simulink model "pmsm_with_fuel_cell"  (R2024b)
settings: Solver=ode14x  StartTime=0.0  StopTime=1  MaxStep=2e-6  RelTol=1e-3
InitFcn:
  | % Control parameters
  | Ts = 2e-6;   % Fundamental sample time
  | fsw = 2e3;   % Switching frequency (Hz)
  | fc = fsw*10; % Control loop frequency (Hz)
  | Tsc = 1/fc;  % Control loop sample time
  | 
  | % PMSM parameters
  | PM = 0.03; % Permanent magnet flux linkage
  | Ld = 2e-4;  % d-axis inductance
  | Lq = 2e-4;  % q-axis inductance
  | L0 = 2e-4;  % 0-axis inductance
  | Rs = 0.013; % Stator resistance
  | N = 6; % Number of pole pairs
  | J = 0.2; % Moment of inertia
  | 
  | % Operating and derived limits
  | Imax = 100;  % Max stator current (peak value)
  | Tmax = 1.5*N*PM*Imax; % Max lectromagnetic torque
  | fnom = 100;  % Nominal frequency (Hz)
  | rpm_nom = 60*fnom/N;      % Nominal rotor speed (rpm)
  | omegam_nom = 2*pi*fnom/N; % Nominal mechanical rotor speed
  | Pmax = omegam_nom*Tmax;     % Maximum power
libraries: fl_lib x27, nesl_utility x24, ee_lib x18, batteryecm_lib x1, eePmsmFieldOrientedControl x1, rllib x1
(part 1 of 2)
settings Model: SimulationMode=accelerator  Creator=pruth  LastModifiedBy=pruth
settings SolverCC: ExtrapolationOrder=2
settings DebuggingCC: SignalInfNanChecking=error
settings SimscapeCC: SimscapeLogType=all

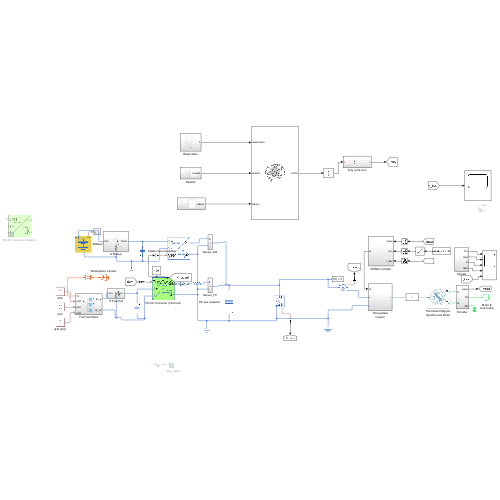
[thumbnail: Simulink's stored preview of the top-level diagram]
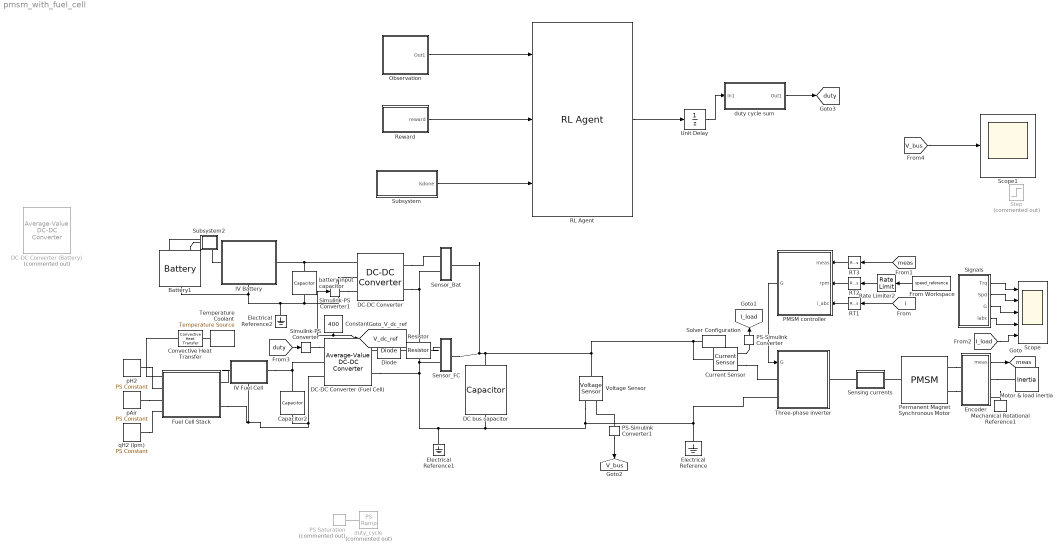
== system pmsm_with_fuel_cell ==
  Battery1 : batteryecm_lib/Battery  Vnom=400 V  prm_dir=1  R1_dis=2 Ohm  R1_ch=2 Ohm  R1=0.05 Ohm  prm_AH=2  AH=30 hr*A  V1=330 V  AH1=15 hr*A  prm_R2=1  R2=2000 Ohm  Tmeas=298.15 K  charge_measurement_port=simscape.enum.battery.enable.yes  prm_dyn=1  Rp1=0.005 Ohm  tau1=30 s  Rp2=0.005 Ohm  tau2=30 s  Rp3=0.005 Ohm  tau3=30 s  Rp4=0.005 Ohm  tau4=30 s  Rp5=0.005 Ohm  tau5=30 s  prm_fade=simscape.enum.battery.prm_fade.enabled  N_fade=10000  AH_fade=29.7 hr*A  R1_fade=0.0505 Ohm  R1_ch_fade=2.02 Ohm  V1_fade=329 V  prm_age=1  prm_age_OCV=1  OCV_age=0.9  SOC_age=60  Tmeas_age=298.15 K  delta_time_age_vec=[0] d  temperature_age_vec=[273] K  OCV_scaling_age=2.2134e6  OCV_offset_age=1.632e6  temp_exp_age=0.515833569 V  t_exp_age=0.75  Vnom_T2=12 V  R1_T2=2.2 Ohm  R1_T2_dis=2.2 Ohm  R1_T2_ch=2.2 Ohm  V1_T2=11.4 V  R2_T2=2200 Ohm  Rp1_T2=0.005 Ohm  tau1_T2=30 s  Rp2_T2=0.005 Ohm  tau2_T2=30 s  Rp3_T2=0.005 Ohm  tau3_T2=30 s  Rp4_T2=0.005 Ohm  tau4_T2=30 s  Rp5_T2=0.005 Ohm  tau5_T2=30 s  Tmeas2=273.15 K  thermal_port=simscape.enum.thermaleffects.omit  thermal_mass=30000 J/K  i_specify=off  i_priority=None  i=0 A  i_nominal_specify=off  i_nominal_value=1  i_nominal_unit=A  v_specify=on  v_priority=Low  v=330 V  v_nominal_specify=off  v_nominal_value=1  v_nominal_unit=V  charge_specify=on  charge_priority=High  charge=15 hr*A  charge_nominal_specify=off  charge_nominal_value=1  charge_nominal_unit=hr*A  num_cycles_specify=on  num_cycles_priority=High  num_cycles=10  num_cycles_nominal_specify=off  num_cycles_nominal_value=1  num_cycles_nominal_unit=1  temperature_specify=off  temperature_priority=High  temperature=298.15 K  temperature_nominal_specify=off  temperature_nominal_value=1  temperature_nominal_unit=K
      settings: LogSimulationData=on  InternalSimscapePortConfiguration="{\"Bottom\":[],\"Left\":[{\"id\":\"p\",\"label\":\"+\",\"type\":\"foundation.electrical.electrical\"},{\"id\":\"q\",\"label\":\"q\",\"type\":\"output\"}],\"Right\":[{\"id\":\"n\",\"label\":\"-\",\"type\":\"foundation.electrical.electrical\"}],\"Top\":[]}"
  Capacitor2 : fl_lib/Electrical/Electrical Elements/Capacitor  c=1e-3 F  r=1e-3 Ohm  g=0 1/Ohm  i_specify=off  i_priority=None  i=0 A  i_nominal_specify=off  i_nominal_value=1  i_nominal_unit=A  v_specify=off  v_priority=None  v=0 V  v_nominal_specify=off  v_nominal_value=1  v_nominal_unit=V  vc_specify=on  vc_priority=Low  vc=650 V  vc_nominal_specify=off  vc_nominal_value=1  vc_nominal_unit=V
  Constant : Constant  Value=400
  Convective Heat Transfer : fl_lib/Thermal/Thermal Elements/Convective Heat Transfer  thermal_type=foundation.enum.constant_variable.constant  area=300 cm^2  heat_tr_coeff=75 W/(m^2 * K)  min_heat_tr_coeff=1e-3 W/(K*m^2)  T_specify=off  T_priority=None  T=0 K  T_nominal_specify=off  T_nominal_value=1  T_nominal_unit=K  Q_specify=off  Q_priority=None  Q=0 W  Q_nominal_specify=off  Q_nominal_value=1  Q_nominal_unit=W
  Current Sensor : fl_lib/Electrical/Electrical Sensors/Current Sensor
  DC bus capacitor : fl_lib/Electrical/Electrical Elements/Capacitor  c=5 mF  r=1e-3 Ohm  g=0 1/Ohm  i_specify=off  i_priority=None  i=0 A  i_nominal_specify=off  i_nominal_value=1  i_nominal_unit=A  v_specify=off  v_priority=Low  v=400 V  v_nominal_specify=off  v_nominal_value=1  v_nominal_unit=V  vc_specify=on  vc_priority=High  vc=400 V  vc_nominal_specify=off  vc_nominal_value=1  vc_nominal_unit=V
  DC-DC Converter : ee_lib/Semiconductors & Converters/Converters/DC-DC Converter  Vref_option=ee.enum.converters.voltageref.external  v_ref=10 V  P_rated=10000 W  droop_enabled=true  droop_param=ee.enum.converters.droop.value  droop=0.15 V/A  droop_percent=2  Vref_droop=400 V  reversible=ee.enum.converters.directionality.bidirectional  G_diode=1e-8 1/Ohm  P_fixed=0.5 W  losses_option=ee.enum.converters.lossesOption.proportionalToSquaredCurrent  eff_rated=98  tableOption=ee.enum.converters.lossTableOptionThermal.currentTemp  i_eff_vec=[-2, -1, 1, 2] A  v_eff_vec=[15, 30, 45] V  eff_vec=[66, 76, 80, 74]  eff_2D_table=[66, 66, 66; 76, 76, 76; 80, 80, 80; 74, 74, 74]  model_dynamics=ee.enum.converters.dynamics.no  tau=0.005 s  v_ini=400 V  v1_min=1 V  R1=1000 Ohm  R2=1000 Ohm  fault_condition=ee.enum.faults.faultInputCondition.greaterThan  fault_threshold=0.5  T_eff_vec=[280, 300, 320] K  eff_3D_table=repmat([66; 76; 80; 74], 1, 3, 3)  thermal_mass=100 J/K  initial_temperature=298.15 K
      settings: InternalSimscapePortConfiguration="{\"Bottom\":[],\"Left\":[{\"id\":\"p1\",\"label\":\"1+\",\"type\":\"foundation.electrical.electrical\"},{\"id\":\"n1\",\"label\":\"1-\",\"type\":\"foundation.electrical.electrical\"},{\"id\":\"Vref\",\"label\":\"Vref\",\"type\":\"input\"}],\"Right\":[{\"id\":\"p2\",\"label\":\"2+\",\"type\":\"foundation.electrical.electrical\"},{\"id\":\"n2\",\"label\":\"2-\",\"type\":\"foundation.electrical.electrical\"}],\"Top\":[]}"
  DC-DC Converter (Battery) : ee_lib/Semiconductors & Converters/Converters/Average-Value DC-DC Converter  Commented=on  control_option=ee.enum.converters.controlinput.voltage  converter_type=ee.enum.converters.dcdctype.boost  efficiency_option=ee.enum.converters.efficiency.constant  efficiency_fixed=100  i_vec=[0, 2, 5] A  efficiency_vec=[90, 95, 98]
      settings: LogSimulationData=on  InternalSimscapePortConfiguration="{\"Bottom\":[],\"Left\":[{\"id\":\"Vref\",\"label\":\"Vref\",\"type\":\"input\"},{\"id\":\"p1\",\"label\":\"1+\",\"type\":\"foundation.electrical.electrical\"},{\"id\":\"n1\",\"label\":\"1-\",\"type\":\"foundation.electrical.electrical\"}],\"Right\":[{\"id\":\"p2\",\"label\":\"2+\",\"type\":\"foundation.electrical.electrical\"},{\"id\":\"n2\",\"label\":\"2-\",\"type\":\"foundation.electrical.electrical\"}],\"Top\":[]}"
  DC-DC Converter (Fuel Cell) : ee_lib/Semiconductors & Converters/Converters/Average-Value DC-DC Converter  control_option=ee.enum.converters.controlinput.dutycycle  converter_type=ee.enum.converters.dcdctype.buck  efficiency_option=ee.enum.converters.efficiency.constant  efficiency_fixed=100  i_vec=[0, 2, 5] A  efficiency_vec=[90, 95, 98]
      settings: LogSimulationData=on  InternalSimscapePortConfiguration="{\"Bottom\":[],\"Left\":[{\"id\":\"DutyCycle\",\"label\":\"DutyCycle\",\"type\":\"input\"},{\"id\":\"p1\",\"label\":\"1+\",\"type\":\"foundation.electrical.electrical\"},{\"id\":\"n1\",\"label\":\"1-\",\"type\":\"foundation.electrical.electrical\"}],\"Right\":[{\"id\":\"p2\",\"label\":\"2+\",\"type\":\"foundation.electrical.electrical\"},{\"id\":\"n2\",\"label\":\"2-\",\"type\":\"foundation.electrical.electrical\"}],\"Top\":[]}"
  Diode : ee_lib/Semiconductors & Converters/Diode  ModelType=ee.enum.diode.modelType.pwl  TableType=ee.enum.diode.tableType.IfMat  IfMat=[.07, .12, .19, 1.75, 4.24, 7.32, 11.2; .16, .3, .72, 2.14, 5.02, 8.35, 13.12] A  VfMat=[.9, 1.15, 1.25, 1.5, 1.75, 2.17, 2.6, 2.85; .58, .68, .75, 1.1, 1.38, 1.77, 2.27, 2.7] V  TjVec=[25, 125] degC  VfVec=[.5, .7, .9, 1.3, 1.7, 2.1, 2.5] V  IfVec=[.1, .2, .5, 1, 2, 4, 7, 10] A  IrMat=[1e-06, 2e-06, 5e-06, 1e-05, 2.5e-05, 5e-05, .0001; 2e-06, 5e-06, 1e-05, 4e-05, 8e-05, .0002, .0005] A  VrMat=[10, 100, 200, 250, 300, 325, 350; 10, 70, 160, 220, 270, 300, 320] V  VrVec=[10, 20, 40, 50, 70, 80, 100] V  IrVec=[1e-06, 2e-06, 5e-06, 1e-05, 2e-05, 5e-05, .0001] A  Vf=0.8 V  Ron=0.001 Ohm  Goff=1e-8 S  prmExp=ee.enum.diode.expParam.useTwo  I12=[.0137, .545] A  V12=[.6, .7] V  RS=0 Ohm  Tmeas=298.15 K  IS=1e-12 A  ec=1  I1=0.0137 A  V1=0.6 V  N_series=1  N_parallel=1  ZenerEnable=false  Rz=0.3 Ohm  BV=inf V  C_param=ee.enum.diode.capParam.fixed  CJ=0 pF  CJ0=5 pF  Vvec=[.1, 10, 100] V  Cvec=[3.5, 1, .4] pF  VJ=1 V  Mgrad=0.5  FC=0.5  Q_param=ee.enum.diode.recoveryParam.off  iRM=-7.15 A  iF=4 A  didt=-750 A/us  trr_factor=3  trr=115 ns  Qrr=150 nA*s  Vr=-600 V  Ls=150 nH  Erec=0.03 J  TT=50 ns  tau=100 ns  T_param=ee.enum.diode.temperatureParam.off  Tdevice=298.15 K  I1_T2=0.245 A  V1_T2=0.5 V  IS_T2=1.25e-7 A  Tmeas2=125 degC  XTI_param=ee.enum.diode.xtiParam.pn  XTI=3  EG_param=ee.enum.diode.egapParam.material_si  EG=1.11 eV  dBVdT=0 V/K  fault_action=simscape.enum.assert.action.none  t_fault=inf s  enable_fault_input=simscape.enum.onoff.off  i_specify=off  i_priority=None  i=0 A  i_nominal_specify=off  i_nominal_value=1  i_nominal_unit=A  v_specify=off  v_priority=None  v=0 V  v_nominal_specify=off  v_nominal_value=1  v_nominal_unit=V  v_capacitor_specify=off  v_capacitor_priority=None  v_capacitor=0 V  v_capacitor_nominal_specify=off  v_capacitor_nominal_value=1  v_capacitor_nominal_unit=V  Qj_specify=off  Qj_priority=High  Qj=0 C  Qj_nominal_specify=off  Qj_nominal_value=1  Qj_nominal_unit=C  i_diode_specify=off  i_diode_priority=None  i_diode=0 A  i_diode_nominal_specify=off  i_diode_nominal_value=1  i_diode_nominal_unit=A  v_diode_specify=off  v_diode_priority=None  v_diode=0 V  v_diode_nominal_specify=off  v_diode_nominal_value=1  v_diode_nominal_unit=V  i_capacitor_specify=off  i_capacitor_priority=None  i_capacitor=0 A  i_capacitor_nominal_specify=off  i_capacitor_nominal_value=1  i_capacitor_nominal_unit=A  power_dissipated_specify=off  power_dissipated_priority=None  power_dissipated=0 W  power_dissipated_nominal_specify=off  power_dissipated_nominal_value=1  power_dissipated_nominal_unit=W  fidelity_level=ee.enum.diode.fidelity.idealSwitch  rec_loss_model=ee.enum.diode.reverseRecoveryModel.fixed  ErecVal=0 J  scaleWithIandV=true  ErecMat=zeros(2, 3) J  TjrecVec=[298.15, 398.15] K  IfrecVec=[.1, 1, 10] A  IrecVal=10 A  VrecVal=10 V  tFilter=1 / 1000 / 100 s  thermal_network_parameterization=ee.enum.thermalNetworkTopology.junctionCase  Rth=[0, 10] K/W  Rth_Cauer=[1, 3, 10] K/W  Rth_Foster=[.08, .14, .22, .16] K/W  thermal_mass_parameterization=ee.enum.thermalNetwork.timeconstant  thermal_mass=[0, 1] J/K  thermal_mass_Cauer=[.1, .3, 1] J/K  thermal_mass_Foster=[.001, .005, .05, .5] J/K  thermal_time_constant=[0, 10] s  thermal_time_constant_Cauer=[1, 3, 10] s  thermal_time_constant_Foster=[7e-05, .0007, .01, .08] s  thermal_mass_initial_temperatures=[25, 25] degC  thermal_mass_initial_temperatures_Cauer=[25, 25, 25] degC  junction_thermal_mass=0.01 J/K  Tvec_initial_Foster=[25, 25, 25, 25] degC  no_thermal_network=1  junction_temperature_specify=off  junction_temperature_priority=None  junction_temperature=25 degC  junction_temperature_nominal_specify=off  junction_temperature_nominal_value=1  junction_temperature_nominal_unit=degC
  Electrical Reference : fl_lib/Electrical/Electrical Elements/Electrical Reference
  Electrical Reference1 : fl_lib/Electrical/Electrical Elements/Electrical Reference
  Electrical Reference2 : fl_lib/Electrical/Electrical Elements/Electrical Reference
  Encoder : Subsystem
  From Workspace : FromWorkspace  VariableName=speed_reference
  Fuel Cell Stack : Subsystem
  IV Battery : Subsystem
      settings: PortSchema="{\"entries\":[{\"content\":{\"sides\":[{\"content\":{\"connectorIds\":[\"LConn1\"]},\"type\":\"ConnectorPlacement.EquallySpacedRectSide\",\"uuid\":\"c74c3ffe-4181-439f-8f63-47f39e558e2a\"},{\"content\":{\"connectorIds\":[\"RConn1\"],\"side\":\"RIGHT\"},\"type\":\"ConnectorPlacement.EquallySpacedRectSide\",\"uuid\":\"9438a85a-aa2d-46a8-960b-411a29715dec\"},{\"content\":{\"side\":\"TOP\"},\"type\":\"ConnectorPlacement.EquallySpacedRectSide\",\"uuid\":\"d1231007-950c-459e-80d3-fa3ee648e50c\"},{\"content\":{\"connectorIds\":[\"RConn2\"],\"side\":\"BOTTOM\"},\"type\":\"ConnectorPlacement.EquallySpacedRectSide\",\"uuid\":\"ff976e01-1be4-46b4-8cbd-cb7b347558a5\"}]},\"type\":\"ConnectorPlacement.EquallySpacedConnector\",\"uuid\":\"65ee485a-61b0-4423-8d03-0ee370ce5677\"}],\"packageUris\":[\"http://schema.mathworks.com/mf0/Connector/R2020b\"],\"version\":\"1.0\"}"
  IV Fuel Cell : Subsystem
      settings: PortSchema="{\"entries\":[{\"content\":{\"sides\":[{\"content\":{\"connectorIds\":[\"LConn1\"]},\"type\":\"ConnectorPlacement.EquallySpacedRectSide\",\"uuid\":\"c74c3ffe-4181-439f-8f63-47f39e558e2a\"},{\"content\":{\"connectorIds\":[\"RConn1\"],\"side\":\"RIGHT\"},\"type\":\"ConnectorPlacement.EquallySpacedRectSide\",\"uuid\":\"9438a85a-aa2d-46a8-960b-411a29715dec\"},{\"content\":{\"side\":\"TOP\"},\"type\":\"ConnectorPlacement.EquallySpacedRectSide\",\"uuid\":\"d1231007-950c-459e-80d3-fa3ee648e50c\"},{\"content\":{\"connectorIds\":[\"RConn2\"],\"side\":\"BOTTOM\"},\"type\":\"ConnectorPlacement.EquallySpacedRectSide\",\"uuid\":\"02f3766e-517b-4ca7-9ef5-b22112c4fb5b\"}]},\"type\":\"ConnectorPlacement.EquallySpacedConnector\",\"uuid\":\"65ee485a-61b0-4423-8d03-0ee370ce5677\"}],\"packageUris\":[\"http://schema.mathworks.com/mf0/Connector/R2020b\"],\"version\":\"1.0\"}"
  Mechanical Rotational Reference1 : fl_lib/Mechanical/Rotational Elements/Mechanical Rotational Reference
  Motor & load inertia : fl_lib/Mechanical/Rotational Elements/Inertia  inertia=J kg*m^2  num_ports=foundation.enum.numPorts2.one  w_specify=on  w_priority=High  w=0 rpm  w_nominal_specify=off  w_nominal_value=1  w_nominal_unit=rad/s  t_specify=off  t_priority=High  t=0 N*m  t_nominal_specify=off  t_nominal_value=1  t_nominal_unit=N*m
  Observation : Subsystem
  PMSM controller : Subsystem
  PS Saturation : fl_lib/Physical Signals/Nonlinear Operators/PS Saturation  Commented=on  upper_limit=0.95  lower_limit=0.15
  PS-Simulink Converter : nesl_utility/PS-Simulink Converter  PhysicalDomain=network_engine_domain  SubClassName=ps_output  LeftPortType=input  RightPortType=output  PseudoPeriodic=off  Frequencies=[]  VectorFormat=inherit  Unit=inherit  AffineConversion=off
  PS-Simulink Converter1 : nesl_utility/PS-Simulink Converter  PhysicalDomain=network_engine_domain  SubClassName=ps_output  LeftPortType=input  RightPortType=output  PseudoPeriodic=off  Frequencies=[]  VectorFormat=inherit  Unit=inherit  AffineConversion=off
  Permanent Magnet Synchronous Motor : ee_lib/Electromechanical/Permanent Magnet/PMSM  port_option=ee.enum.threePhasePort.composite  winding_type=ee.enum.statorconnection.wye  machine_param=ee.enum.pmsm.parameterization.constant  nPolePairs=N  pmflux_param=ee.enum.pmflux.fluxlinkage  pm_flux_linkage=PM Wb  torque_constant=0.18 N*m/A  back_emf_constant=0.18 V/(rad/s)  stator_param=ee.enum.statorparam.LdLqL0  Ld=Ld H  Lq=Lq H  idVec=[-200, 0, 200] A  iqVec=[-200, 0, 200] A  LdMatrix=0.0002 * ones(3, 3) H  LqMatrix=0.0002 * ones(3, 3) H  PmMatrix=0.1 * ones(3, 3) Wb  ktMatrix=0.18 * ones(3, 3) N*m/A  keMatrix=0.18 * ones(3, 3) V/(rad/s)  L0=L0 H  Ls=0.0002 H  Lm=0.00002 H  Ms=0.00002 H  Rs=Rs Ohm  zero_sequence=ee.enum.park.zerosequence.exclude  axes_param=ee.enum.rotorangle.qaxis  loss_param=ee.enum.ironloss.none  losses_oc=[0, 0, 0] W  losses_sc=[0, 0, 0] W  f_losses=60 Hz  Isc_losses=95 A  J=0 kg*m^2  lam=1e-3 N*m/(rad/s)  i_d_specify=off  i_d_priority=None  i_d=0 A  i_d_nominal_specify=off  i_d_nominal_value=1  i_d_nominal_unit=A  i_q_specify=off  i_q_priority=None  i_q=0 A  i_q_nominal_specify=off  i_q_nominal_value=1  i_q_nominal_unit=A  torque_specify=off  torque_priority=None  torque=0 N*m  torque_nominal_specify=off  torque_nominal_value=1  torque_nominal_unit=N*m  angular_velocity_specify=on  angular_velocity_priority=None  angular_velocity=0 rpm  angular_velocity_nominal_specify=off  angular_velocity_nominal_value=1  angular_velocity_nominal_unit=rpm  angular_position_specify=on  angular_position_priority=High  angular_position=0 rad  angular_position_nominal_specify=off  angular_position_nominal_value=1  angular_position_nominal_unit=deg  alpha=3.93e-3 1/K  alpha_flux=-0.001 1/K  Tmeas=298.15 K  stator_thermal_mass=100 J/K  rotor_thermal_mass=200 J/K  Rm_percent_rotor=90  Rd_percent_rotor=30  temperatureA_specify=off  temperatureA_priority=High  temperatureA=25 degC  temperatureA_nominal_specify=off  temperatureA_nominal_value=1  temperatureA_nominal_unit=degC  temperatureB_specify=off  temperatureB_priority=High  temperatureB=25 degC  temperatureB_nominal_specify=off  temperatureB_nominal_value=1  temperatureB_nominal_unit=degC  temperatureC_specify=off  temperatureC_priority=High  temperatureC=25 degC  temperatureC_nominal_specify=off  temperatureC_nominal_value=1  temperatureC_nominal_unit=degC  temperatureR_specify=off  temperatureR_priority=High  temperatureR=25 degC  temperatureR_nominal_specify=off  temperatureR_nominal_value=1  temperatureR_nominal_unit=degC
      settings: InternalSimscapePortConfiguration="{\"Bottom\":[],\"Left\":[{\"id\":\"N\",\"label\":\"~\",\"type\":\"foundation.electrical.three_phase\"}],\"Right\":[{\"id\":\"R\",\"label\":\"R\",\"type\":\"foundation.mechanical.rotational.rotational\"},{\"id\":\"C\",\"label\":\"C\",\"type\":\"foundation.mechanical.rotational.rotational\"}],\"Top\":[]}"
  RL Agent : rllib/RL Agent  Agent=agent  ExternalActionAsInput=off  ProvideLastAction=off  ProvideCumRwd=off  TreatAsDirectFeedthrough=on  UseStrictObservationDataTypes=off
  RT1 : RateTransition  OutPortSampleTime=Tsc
  RT2 : RateTransition  OutPortSampleTime=Tsc
  RT3 : RateTransition  OutPortSampleTime=Tsc
  Rate Limiter2 : RateLimiter  RisingSlewLimit=8000  FallingSlewLimit=-8000  SampleTimeMode=inherited
  Resistor : fl_lib/Electrical/Electrical Elements/Resistor  R=0.1 Ohm  i_specify=off  i_priority=None  i=0 A  i_nominal_specify=off  i_nominal_value=1  i_nominal_unit=A  v_specify=off  v_priority=None  v=0 V  v_nominal_specify=off  v_nominal_value=1  v_nominal_unit=V
  Reward : Subsystem
  Scope : Scope  NumInputPorts=5
  Scope1 : Scope
  Sensing currents : Subsystem
      mask Display: disp('i')
  Sensor_Bat : Subsystem
  Sensor_FC : Subsystem
  "Signals " : Subsystem
  Simulink-PS Converter : nesl_utility/Simulink-PS Converter  PhysicalDomain=network_engine_domain  SubClassName=ps_input  LeftPortType=input  RightPortType=output  PseudoPeriodic=off  Frequencies=[]  NoiseDistribution=none  NoiseParameters=[]  Unit=1  AffineConversion=off  FilteringAndDerivatives=filter  SimscapeFilterOrder=2  InputFilterTimeConstant=1e-5  UdotUserProvided=0
  Simulink-PS Converter1 : nesl_utility/Simulink-PS Converter  PhysicalDomain=network_engine_domain  SubClassName=ps_input  LeftPortType=input  RightPortType=output  PseudoPeriodic=off  Frequencies=[]  NoiseDistribution=none  NoiseParameters=[]  Unit=1  AffineConversion=off  FilteringAndDerivatives=provide  SimscapeFilterOrder=1  InputFilterTimeConstant=0.001  UdotUserProvided=0
  Solver Configuration : nesl_utility/Solver Configuration  PhysicalDomain=network_engine_domain  SubClassName=solver  LeftPortType=input  RightPortType=generic  Tones=[]  Harmonics=[]  SimulateNoise=off  Profile=off  UseLocalSampling=off  EnableSwitchedLinearOptims=on  FrequencyDomain=off  UseCCode=off  RelTol=0.001  AbsTol=1e-06  MinStep=1e-09  ToWorkspace=off  RevertToSquareIcSolve=off  NumHomotopyIterations=100  PhasorMode=off  PhasorModeNumHarmonics=1  ConsistencySolver=NEWTON_FTOL  IndexReductionMethod=DerivativeReplacement  DoDC=off  ResidualTolerance=1e-3  ConsistencyTolSource=GLOBAL  ConsistencyAbsTol=0.001  ConsistencyRelTol=0.001  ConsistencyTolFactor=0.001  UseLocalSolver=on  LocalSolverChoice=NE_BACKWARD_EULER_ADVANCER  ResolveIndetEquations=on  FunctionEvalNumThread=1  LocalSolverSampleTime=Ts  DoFixedCost=on  MaxNonlinIter=4  MaxModeIter=2  ComputeImpulses=off  ImpulseIterations=2  LinearAlgebra=auto  LinearAlgebraNumThread=0  EquationFormulation=NE_TIME_EF  DelaysMemoryBudget=1024  AutomaticFiltering=on  FilteringTimeConstant=0.001  PartitionStorageMethod=AS_NEEDED  PartitionMemoryBudget=1024  PartitionMethod=FAST  MultibodyUseLocalSolver=off  MultibodyLocalSolverChoice=ODE1  MultibodyLocalSolverSampleTime=0.001
  Step : Step  Commented=on  Time=0.1  After=500  SampleTime=0
  Subsystem : Subsystem
  Subsystem2 : Subsystem
  Temperature Coolant : fl_lib/Thermal/Thermal Sources/Temperature Source  temperature=293.15 K
  Three-phase inverter : Subsystem
  Unit Delay : UnitDelay  SampleTime=-1  HasFrameUpgradeWarning=on
  Voltage Sensor : fl_lib/Electrical/Electrical Sensors/Voltage Sensor
  battery input capacitor : fl_lib/Electrical/Electrical Elements/Capacitor  c=0.1 F  r=1e-3 Ohm  g=0 1/Ohm  i_specify=off  i_priority=None  i=0 A  i_nominal_specify=off  i_nominal_value=1  i_nominal_unit=A  v_specify=off  v_priority=None  v=0 V  v_nominal_specify=off  v_nominal_value=1  v_nominal_unit=V  vc_specify=on  vc_priority=Low  vc=330 V  vc_nominal_specify=off  vc_nominal_value=1  vc_nominal_unit=V
  duty cycle sum : Subsystem
  duty_cycle : fl_lib/Physical Signals/Sources/PS Ramp  Commented=on  slope=-0.8/60 1/s  start_time=0 s  initial_output=0.95
  pAir : fl_lib/Physical Signals/Sources/PS Constant  constant=1 bar
  pH2 : fl_lib/Physical Signals/Sources/PS Constant  constant=5.0 bar
  qH2 (lpm) : fl_lib/Physical Signals/Sources/PS Constant  constant=80 lpm
  tag scope: I_load=global, V_bus=global, V_dc_ref=global, duty=global, meas=global
  wires:
  PS-Simulink Converter/1 -> [I_load]
  [I_load] -> Scope/5
  [i] -> RT1/1
  "Signals "/4(Iabc) -> Scope/4
  RT2/1 -> PMSM controller/2(rpm)
  RT1/1 -> PMSM controller/3(i_abc)
  "Signals "/2(Spd) -> Scope/2
  "Signals "/1(Trq) -> Scope/1
  "Signals "/3(G) -> Scope/3
  RT3/1 -> PMSM controller/1(meas)
  [meas] -> RT3/1
  Encoder/1(meas) -> [meas]
  PMSM controller/1(G) -> Three-phase inverter/1(G)
  PS-Simulink Converter1/1 -> [V_bus]
  Observation/1(Out1) -> RL Agent/1
  duty cycle sum/1(Out1) -> [duty]
  Reward/1(reward) -> RL Agent/2
  Subsystem/1(isdone) -> RL Agent/3
  RL Agent/1 -> Unit Delay/1
  Unit Delay/1 -> duty cycle sum/1(In1)
  Rate Limiter2/1 -> RT2/1
  [duty] -> Simulink-PS Converter/1
  From Workspace/1 -> Rate Limiter2/1
  Constant/1 -> Simulink-PS Converter1/1, [V_dc_ref]
  [V_bus] -> Scope1/1
  connections:
  Sensor_FC/LConn2 -- DC-DC Converter/RConn2 -- Sensor_Bat/LConn2 -- Electrical Reference1/LConn1 -- Voltage Sensor/RConn2 -- Three-phase inverter/LConn2 -- Electrical Reference/LConn1 -- DC bus capacitor/RConn1 -- DC-DC Converter (Fuel Cell)/RConn2
  Sensor_FC/RConn1 -- Voltage Sensor/LConn1 -- Current Sensor/LConn1 -- Solver Configuration/RConn1 -- DC bus capacitor/LConn1 -- Sensor_Bat/RConn1
  Permanent Magnet Synchronous Motor/RConn1 -- Encoder/LConn1
  Current Sensor/RConn2 -- Three-phase inverter/LConn1
  Current Sensor/RConn1 -- PS-Simulink Converter/LConn1
  Mechanical Rotational Reference1/LConn1 -- Encoder/RConn2
  Permanent Magnet Synchronous Motor/LConn1 -- Sensing currents/RConn1
  Encoder/RConn1 -- Motor & load inertia/LConn1
  Permanent Magnet Synchronous Motor/RConn2 -- Encoder/LConn2
  Sensing currents/LConn1 -- Three-phase inverter/RConn1
  Convective Heat Transfer/LConn1 -- Fuel Cell Stack/LConn1
  pAir/RConn1 -- Fuel Cell Stack/LConn3
  duty_cycle/RConn1 -- PS Saturation/LConn1
  pH2/RConn1 -- Fuel Cell Stack/LConn2
  Temperature Coolant/LConn1 -- Convective Heat Transfer/RConn1
  qH2 (lpm)/RConn1 -- Fuel Cell Stack/LConn4
  Subsystem2/LConn1 -- Battery1/LConn2
  PS-Simulink Converter1/LConn1 -- Voltage Sensor/RConn1
  Battery1/LConn1 -- IV Battery/LConn1
  Battery1/RConn1 -- Electrical Reference2/LConn1 -- DC-DC Converter/LConn2 -- battery input capacitor/RConn1 -- IV Battery/RConn2
  battery input capacitor/LConn1 -- IV Battery/RConn1 -- DC-DC Converter/LConn1
  IV Fuel Cell/RConn1 -- DC-DC Converter (Fuel Cell)/LConn2 -- Capacitor2/LConn1
  Fuel Cell Stack/RConn2 -- Capacitor2/RConn1 -- DC-DC Converter (Fuel Cell)/LConn3 -- IV Fuel Cell/RConn2
  Simulink-PS Converter/RConn1 -- DC-DC Converter (Fuel Cell)/LConn1
  IV Fuel Cell/LConn1 -- Fuel Cell Stack/RConn1
  Resistor/RConn1 -- Sensor_FC/LConn1
  Diode/LConn1 -- DC-DC Converter (Fuel Cell)/RConn1
  Diode/RConn1 -- Resistor/LConn1
  DC-DC Converter/RConn1 -- Sensor_Bat/LConn1
  Simulink-PS Converter1/RConn1 -- DC-DC Converter/LConn3

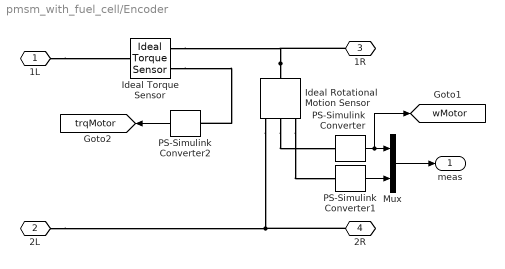
== system pmsm_with_fuel_cell/Encoder ==
  Ideal Rotational Motion Sensor : fl_lib/Mechanical/Mechanical Sensors/Ideal Rotational Motion Sensor  reference=foundation.enum.MeasurementReference.difference  acceleration_port=false  velocity_port=true  position_port=true  wrap_angle=simscape.enum.onoff.off  offset=0 deg
  Ideal Torque Sensor : fl_lib/Mechanical/Mechanical Sensors/Ideal Torque Sensor
  Mux : Mux  Inputs=2
  PS-Simulink Converter : nesl_utility/PS-Simulink Converter  PhysicalDomain=network_engine_domain  SubClassName=ps_output  LeftPortType=input  RightPortType=output  PseudoPeriodic=off  Frequencies=[]  VectorFormat=1-D array  Unit=rad/s  AffineConversion=off
  PS-Simulink Converter1 : nesl_utility/PS-Simulink Converter  PhysicalDomain=network_engine_domain  SubClassName=ps_output  LeftPortType=input  RightPortType=output  PseudoPeriodic=off  Frequencies=[]  VectorFormat=1-D array  Unit=rad  AffineConversion=off
  PS-Simulink Converter2 : nesl_utility/PS-Simulink Converter  PhysicalDomain=network_engine_domain  SubClassName=ps_output  LeftPortType=input  RightPortType=output  PseudoPeriodic=off  Frequencies=[]  VectorFormat=1-D array  Unit=N*m  AffineConversion=off
  1L : PMIOPort  Side=Left
  2L : PMIOPort  Port=2  Side=Left
  1R : PMIOPort  Port=3  Side=Right
  2R : PMIOPort  Port=4  Side=Right
  meas : Outport  VectorParamsAs1DForOutWhenUnconnected=off
  tag scope: trqMotor=global, wMotor=global
  wires:
  PS-Simulink Converter2/1 -> [trqMotor]
  Mux/1 -> meas/1
  PS-Simulink Converter1/1 -> Mux/2
  PS-Simulink Converter/1 -> [wMotor], Mux/1
  connections:
  Ideal Torque Sensor/RConn2 -- PS-Simulink Converter2/LConn1
  1L/RConn1 -- Ideal Torque Sensor/LConn1
  2R/RConn1 -- 2L/RConn1 -- Ideal Rotational Motion Sensor/RConn1
  Ideal Rotational Motion Sensor/LConn1 -- 1R/RConn1 -- Ideal Torque Sensor/RConn1
  Ideal Rotational Motion Sensor/RConn2 -- PS-Simulink Converter/LConn1
  Ideal Rotational Motion Sensor/RConn3 -- PS-Simulink Converter1/LConn1

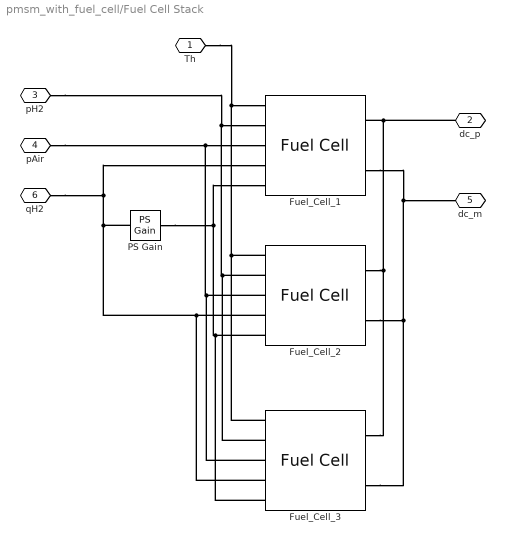
== system pmsm_with_fuel_cell/Fuel Cell Stack ==
  Fuel_Cell_1 : ee_lib/Sources/Fuel Cell  model_fidelity=ee.enum.fuelcell.fidelity.detailed  Eoc=65 V  A=0.23 V  ri=0.05 Ohm  i0=80 A  i_lim=200 A  N_cell=65  number_unit=10  pH2_nom=1.5e5 Pa  pO2_nom=1.0e5 Pa  xH2=99  xO2=21  xW=1  dyn=ee.enum.include.no  Rd=0.005 Ohm  tau=10 s  Tnom=293.15 K  thermal_mass=30000 J/K  iFC_specify=off  iFC_priority=None  iFC=0 A  iFC_nominal_specify=off  iFC_nominal_value=1  iFC_nominal_unit=A  vFC_specify=off  vFC_priority=None  vFC=0 V  vFC_nominal_specify=off  vFC_nominal_value=1  vFC_nominal_unit=V  temperature_specify=on  temperature_priority=High  temperature=293.15 K  temperature_nominal_specify=off  temperature_nominal_value=1  temperature_nominal_unit=K
      settings: LogSimulationData=on  InternalSimscapePortConfiguration="{\"Bottom\":[],\"Left\":[{\"id\":\"H\",\"label\":\"H\",\"type\":\"foundation.thermal.thermal\"},{\"id\":\"pfuel\",\"label\":\"pfuel\",\"type\":\"input\"},{\"id\":\"pair\",\"label\":\"pair\",\"type\":\"input\"},{\"id\":\"qfuel\",\"label\":\"qfuel\",\"type\":\"input\"},{\"id\":\"qair\",\"label\":\"qair\",\"type\":\"input\"}],\"Right\":[{\"id\":\"p\",\"label\":\"+\",\"type\":\"foundation.electrical.electrical\"},{\"id\":\"n\",\"label\":\"-\",\"type\":\"foundation.electrical.electrical\"}],\"Top\":[]}"
  Fuel_Cell_2 : ee_lib/Sources/Fuel Cell  model_fidelity=ee.enum.fuelcell.fidelity.detailed  Eoc=65 V  A=0.23 V  ri=0.05 Ohm  i0=80 A  i_lim=200 A  N_cell=65  number_unit=10  pH2_nom=1.5e5 Pa  pO2_nom=1.0e5 Pa  xH2=99  xO2=21  xW=1  dyn=ee.enum.include.no  Rd=0.005 Ohm  tau=10 s  Tnom=293.15 K  thermal_mass=30000 J/K  iFC_specify=off  iFC_priority=None  iFC=0 A  iFC_nominal_specify=off  iFC_nominal_value=1  iFC_nominal_unit=A  vFC_specify=off  vFC_priority=None  vFC=0 V  vFC_nominal_specify=off  vFC_nominal_value=1  vFC_nominal_unit=V  temperature_specify=on  temperature_priority=High  temperature=293.15 K  temperature_nominal_specify=off  temperature_nominal_value=1  temperature_nominal_unit=K
      settings: LogSimulationData=on  InternalSimscapePortConfiguration="{\"Bottom\":[],\"Left\":[{\"id\":\"H\",\"label\":\"H\",\"type\":\"foundation.thermal.thermal\"},{\"id\":\"pfuel\",\"label\":\"pfuel\",\"type\":\"input\"},{\"id\":\"pair\",\"label\":\"pair\",\"type\":\"input\"},{\"id\":\"qfuel\",\"label\":\"qfuel\",\"type\":\"input\"},{\"id\":\"qair\",\"label\":\"qair\",\"type\":\"input\"}],\"Right\":[{\"id\":\"p\",\"label\":\"+\",\"type\":\"foundation.electrical.electrical\"},{\"id\":\"n\",\"label\":\"-\",\"type\":\"foundation.electrical.electrical\"}],\"Top\":[]}"
  Fuel_Cell_3 : ee_lib/Sources/Fuel Cell  model_fidelity=ee.enum.fuelcell.fidelity.detailed  Eoc=65 V  A=0.23 V  ri=0.05 Ohm  i0=80 A  i_lim=200 A  N_cell=65  number_unit=10  pH2_nom=1.5e5 Pa  pO2_nom=1.0e5 Pa  xH2=99  xO2=21  xW=1  dyn=ee.enum.include.no  Rd=0.005 Ohm  tau=10 s  Tnom=293.15 K  thermal_mass=30000 J/K  iFC_specify=off  iFC_priority=None  iFC=0 A  iFC_nominal_specify=off  iFC_nominal_value=1  iFC_nominal_unit=A  vFC_specify=off  vFC_priority=None  vFC=0 V  vFC_nominal_specify=off  vFC_nominal_value=1  vFC_nominal_unit=V  temperature_specify=on  temperature_priority=High  temperature=293.15 K  temperature_nominal_specify=off  temperature_nominal_value=1  temperature_nominal_unit=K
      settings: LogSimulationData=on  InternalSimscapePortConfiguration="{\"Bottom\":[],\"Left\":[{\"id\":\"H\",\"label\":\"H\",\"type\":\"foundation.thermal.thermal\"},{\"id\":\"pfuel\",\"label\":\"pfuel\",\"type\":\"input\"},{\"id\":\"pair\",\"label\":\"pair\",\"type\":\"input\"},{\"id\":\"qfuel\",\"label\":\"qfuel\",\"type\":\"input\"},{\"id\":\"qair\",\"label\":\"qair\",\"type\":\"input\"}],\"Right\":[{\"id\":\"p\",\"label\":\"+\",\"type\":\"foundation.electrical.electrical\"},{\"id\":\"n\",\"label\":\"-\",\"type\":\"foundation.electrical.electrical\"}],\"Top\":[]}"
  PS Gain : fl_lib/Physical Signals/Functions/PS Gain  gain=3
  Th : PMIOPort  Side=Left
  dc_p : PMIOPort  Port=2  Side=Right
  pH2 : PMIOPort  Port=3  Side=Left
  pAir : PMIOPort  Port=4  Side=Left
  dc_m : PMIOPort  Port=5  Side=Right
  qH2 : PMIOPort  Port=6  Side=Left
  connections:
  Fuel_Cell_1/RConn2 -- Fuel_Cell_3/RConn2 -- Fuel_Cell_2/RConn2 -- dc_m/RConn1
  Fuel_Cell_1/RConn1 -- dc_p/RConn1 -- Fuel_Cell_3/RConn1 -- Fuel_Cell_2/RConn1
  pH2/RConn1 -- Fuel_Cell_1/LConn2 -- Fuel_Cell_3/LConn2 -- Fuel_Cell_2/LConn2
  PS Gain/RConn1 -- Fuel_Cell_1/LConn5 -- Fuel_Cell_3/LConn5 -- Fuel_Cell_2/LConn5
  Fuel_Cell_3/LConn4 -- Fuel_Cell_2/LConn4 -- PS Gain/LConn1 -- Fuel_Cell_1/LConn4 -- qH2/RConn1
  pAir/RConn1 -- Fuel_Cell_1/LConn3 -- Fuel_Cell_3/LConn3 -- Fuel_Cell_2/LConn3
  Th/RConn1 -- Fuel_Cell_3/LConn1 -- Fuel_Cell_2/LConn1 -- Fuel_Cell_1/LConn1

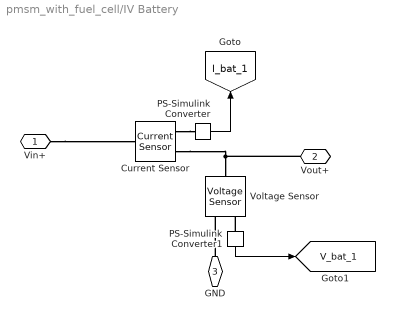
== system pmsm_with_fuel_cell/IV Battery ==
  Current Sensor : fl_lib/Electrical/Electrical Sensors/Current Sensor
  PS-Simulink Converter : nesl_utility/PS-Simulink Converter  PhysicalDomain=network_engine_domain  SubClassName=ps_output  LeftPortType=input  RightPortType=output  PseudoPeriodic=off  Frequencies=[]  VectorFormat=inherit  Unit=inherit  AffineConversion=off
  PS-Simulink Converter1 : nesl_utility/PS-Simulink Converter  PhysicalDomain=network_engine_domain  SubClassName=ps_output  LeftPortType=input  RightPortType=output  PseudoPeriodic=off  Frequencies=[]  VectorFormat=inherit  Unit=inherit  AffineConversion=off
  Voltage Sensor : fl_lib/Electrical/Electrical Sensors/Voltage Sensor
  Vin+ : PMIOPort  Side=Left
  Vout+ : PMIOPort  Port=2  Side=Right
  GND : PMIOPort  Port=3  Side=Right
  tag scope: I_bat_1=global, V_bat_1=global
  wires:
  PS-Simulink Converter/1 -> [I_bat_1]
  PS-Simulink Converter1/1 -> [V_bat_1]
  connections:
  Current Sensor/RConn2 -- Vout+/RConn1 -- Voltage Sensor/LConn1
  Vin+/RConn1 -- Current Sensor/LConn1
  GND/RConn1 -- Voltage Sensor/RConn2
  Current Sensor/RConn1 -- PS-Simulink Converter/LConn1
  PS-Simulink Converter1/LConn1 -- Voltage Sensor/RConn1

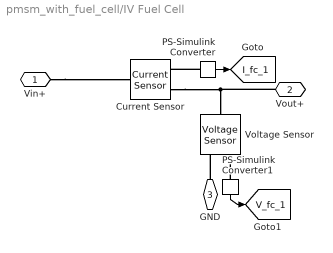
== system pmsm_with_fuel_cell/IV Fuel Cell ==
  Current Sensor : fl_lib/Electrical/Electrical Sensors/Current Sensor
  PS-Simulink Converter : nesl_utility/PS-Simulink Converter  PhysicalDomain=network_engine_domain  SubClassName=ps_output  LeftPortType=input  RightPortType=output  PseudoPeriodic=off  Frequencies=[]  VectorFormat=inherit  Unit=inherit  AffineConversion=off
  PS-Simulink Converter1 : nesl_utility/PS-Simulink Converter  PhysicalDomain=network_engine_domain  SubClassName=ps_output  LeftPortType=input  RightPortType=output  PseudoPeriodic=off  Frequencies=[]  VectorFormat=inherit  Unit=inherit  AffineConversion=off
  Voltage Sensor : fl_lib/Electrical/Electrical Sensors/Voltage Sensor
  Vin+ : PMIOPort  Side=Left
  Vout+ : PMIOPort  Port=2  Side=Right
  GND : PMIOPort  Port=3  Side=Right
  tag scope: I_fc_1=global, V_fc_1=global
  wires:
  PS-Simulink Converter/1 -> [I_fc_1]
  PS-Simulink Converter1/1 -> [V_fc_1]
  connections:
  Current Sensor/RConn2 -- Vout+/RConn1 -- Voltage Sensor/LConn1
  Vin+/RConn1 -- Current Sensor/LConn1
  GND/RConn1 -- Voltage Sensor/RConn2
  PS-Simulink Converter/LConn1 -- Current Sensor/RConn1
  PS-Simulink Converter1/LConn1 -- Voltage Sensor/RConn1

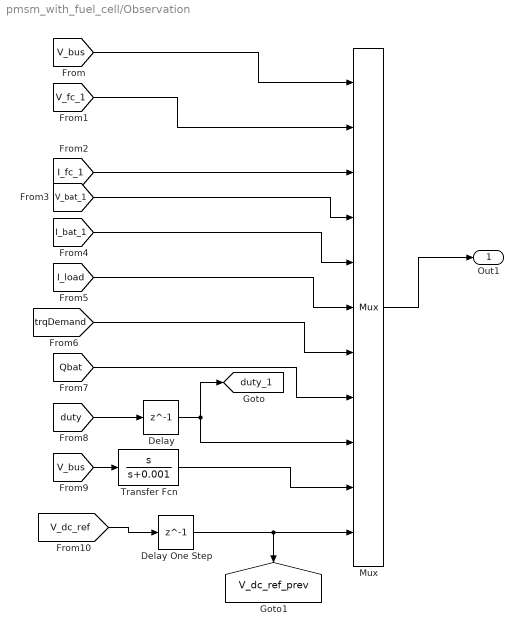
== system pmsm_with_fuel_cell/Observation ==
  Delay : Delay  DelayLength=1  InitialCondition=0.62  SampleTime=Tsc
  Delay One Step : Delay  DelayLength=1
  Mux : Mux  Inputs=11
  Transfer Fcn : TransferFcn  Numerator=[1 0]  Denominator=[1 0.001]
  Out1 : Outport
  tag scope: V_dc_ref_prev=global, duty_1=global
  wires:
  [duty] -> Delay/1
  [V_bus] -> Mux/1
  [V_fc_1] -> Mux/2
  [I_fc_1] -> Mux/3
  [V_bat_1] -> Mux/4
  [I_bat_1] -> Mux/5
  [I_load] -> Mux/6
  [trqDemand] -> Mux/7
  [Qbat] -> Mux/8
  Delay/1 -> [duty_1], Mux/9
  Mux/1 -> Out1/1
  [V_bus] -> Transfer Fcn/1
  Transfer Fcn/1 -> Mux/10
  [V_dc_ref] -> Delay One Step/1
  Delay One Step/1 -> [V_dc_ref_prev], Mux/11

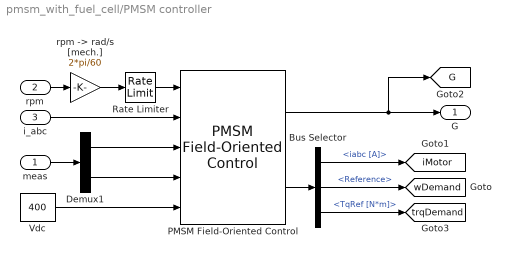
== system pmsm_with_fuel_cell/PMSM controller ==
  meas : Inport
  rpm : Inport  Port=2
  i_abc : Inport  Port=3
  Bus Selector : BusSelector  OutputSignals=iabc [A],Reference,TqRef [N*m]
  Demux1 : Demux  Outputs=2
  PMSM Field-Oriented Control : eePmsmFieldOrientedControl/PMSM Field-Oriented Control  winding_type=Wye-wound  CtrlMode=Velocity control  Vnom=400  Pmax=Pmax  Tmax=Tmax*1.5  p=N  Vdc_on=10  Ts=Ts  Tsc=Tsc  CtrlType=PI control  Kp_w=60  Ki_w=300*2  Kv_w=1  Kaw_w=1000  RefType=Zero d-axis control  rpmVec=[0, 3000]  TqVec=[-100, 0, 100]  VdcVec=[300, 350]  PWMMode=SPWM: sinusoidal PWM  ModFactor=1  idMatrix=zeros(2,3,2)  iqMatrix=zeros(2,3,2)  psim=PM  Ld=0.00024  Lq=0.00029  Rs=0.01  AxisAlignment=Q-axis  Kp_id=0.1  Ki_id=10  Kaw_id=1000  Kp_iq=0.1  Ki_iq=10  Kaw_iq=1000  AxisPrio=Q-axis  ActZC=off  ActFF=on  ParamTypeFF=Constant parameters  LdFF=Ld  LqFF=Lq  psimFF=PM  idVect=[-200, 0, 200]  iqVect=[-200, 0, 200]  LdMatrix=0.0002 * ones(3, 3)  LqMatrix=0.0002 * ones(3, 3)  psimMatrix=0.04 * ones(3, 3)  CPWMMode=SPWM: sinusoidal PWM  fsw=fsw
  Rate Limiter : RateLimiter  RisingSlewLimit=Tmax/J  FallingSlewLimit=-Tmax/J  SampleTimeMode=inherited
  Vdc : Constant  Value=400  SampleTime=Tsc
  "rpm -> rad/s [mech.]" : Gain  Gain=2*pi/60
  G : Outport  VectorParamsAs1DForOutWhenUnconnected=off
  tag scope: G=global, iMotor=global, trqDemand=global, wDemand=global
  wires:
  PMSM Field-Oriented Control/1 -> G/1, [G]
  Vdc/1 -> PMSM Field-Oriented Control/5
  PMSM Field-Oriented Control/2 -> Bus Selector/1
  i_abc/1 -> PMSM Field-Oriented Control/2
  meas/1 -> Demux1/1
  Demux1/1 -> PMSM Field-Oriented Control/3
  Demux1/2 -> PMSM Field-Oriented Control/4
  Bus Selector/1 -> [iMotor]  "<iabc [A]>"
  Bus Selector/2 -> [wDemand]  "<Reference>"
  Bus Selector/3 -> [trqDemand]  "<TqRef [N*m]>"
  rpm/1 -> "rpm -> rad/s [mech.]"/1
  Rate Limiter/1 -> PMSM Field-Oriented Control/1
  "rpm -> rad/s [mech.]"/1 -> Rate Limiter/1

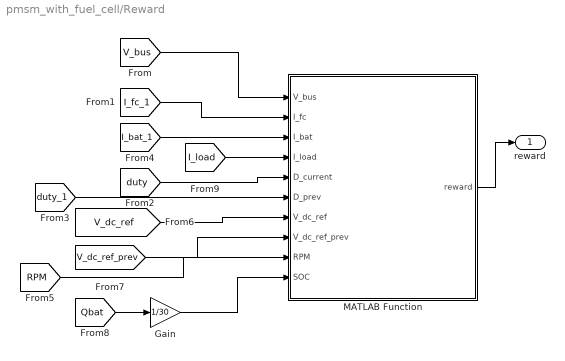
== system pmsm_with_fuel_cell/Reward ==
  Gain : Gain  Gain=1/30
  MATLAB Function : MATLAB Function  TreatAsAtomicUnit=on
  reward : Outport
  wires:
  [V_bus] -> MATLAB Function/1(V_bus)
  [I_fc_1] -> MATLAB Function/2(I_fc)
  [I_bat_1] -> MATLAB Function/3(I_bat)
  [duty] -> MATLAB Function/5(D_current)
  [duty_1] -> MATLAB Function/6(D_prev)
  MATLAB Function/1(reward) -> reward/1
  [RPM] -> MATLAB Function/9(RPM)
  [V_dc_ref] -> MATLAB Function/7(V_dc_ref)
  [V_dc_ref_prev] -> MATLAB Function/8(V_dc_ref_prev)
  [Qbat] -> Gain/1
  Gain/1 -> MATLAB Function/10(SOC)
  [I_load] -> MATLAB Function/4(I_load)

== system pmsm_with_fuel_cell/Sensing currents ==
  Current Sensor : ee_lib/Sensors & Transducers/Current Sensor (Three-Phase)
  Gain : Gain  Commented=through  Gain=1/sqrt(3)
  PS-Simulink Converter : nesl_utility/PS-Simulink Converter  PhysicalDomain=network_engine_domain  SubClassName=ps_output  LeftPortType=input  RightPortType=output  PseudoPeriodic=off  Frequencies=[]  VectorFormat=1-D array  Unit=A  AffineConversion=off
  Conn1 : PMIOPort  Side=Left
  Conn2 : PMIOPort  Port=2  Side=Right
  tag scope: i=global
  wires:
  PS-Simulink Converter/1 -> Gain/1
  Gain/1 -> [i]
  connections:
  Current Sensor/RConn1 -- PS-Simulink Converter/LConn1
  Conn2/RConn1 -- Current Sensor/RConn2
  Current Sensor/LConn1 -- Conn1/RConn1

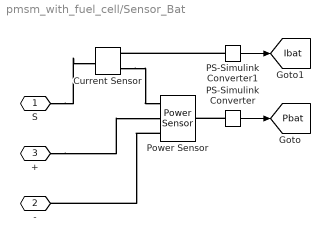
== system pmsm_with_fuel_cell/Sensor_Bat ==
  Current Sensor : fl_lib/Electrical/Electrical Sensors/Current Sensor
  PS-Simulink Converter : nesl_utility/PS-Simulink Converter  PhysicalDomain=network_engine_domain  SubClassName=ps_output  LeftPortType=input  RightPortType=output  PseudoPeriodic=off  Frequencies=[]  VectorFormat=1-D array  Unit=kW  AffineConversion=off
  PS-Simulink Converter1 : nesl_utility/PS-Simulink Converter  PhysicalDomain=network_engine_domain  SubClassName=ps_output  LeftPortType=input  RightPortType=output  PseudoPeriodic=off  Frequencies=[]  VectorFormat=1-D array  Unit=A  AffineConversion=off
  Power Sensor : ee_lib/Sensors & Transducers/Power Sensor  measurement_type=1  averaging_period=1e-4 s
  S : PMIOPort  Side=Left
  - : PMIOPort  Port=2  Side=Left
  + : PMIOPort  Port=3  Side=Right
  tag scope: Ibat=global, Pbat=global
  wires:
  PS-Simulink Converter/1 -> [Pbat]
  PS-Simulink Converter1/1 -> [Ibat]
  connections:
  +/RConn1 -- Power Sensor/LConn2
  Power Sensor/LConn3 -- -/RConn1
  PS-Simulink Converter/LConn1 -- Power Sensor/RConn1
  Current Sensor/RConn2 -- Power Sensor/LConn1
  S/RConn1 -- Current Sensor/LConn1
  PS-Simulink Converter1/LConn1 -- Current Sensor/RConn1

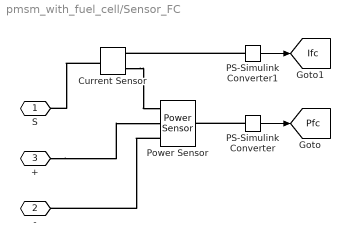
== system pmsm_with_fuel_cell/Sensor_FC ==
  Current Sensor : fl_lib/Electrical/Electrical Sensors/Current Sensor
  PS-Simulink Converter : nesl_utility/PS-Simulink Converter  PhysicalDomain=network_engine_domain  SubClassName=ps_output  LeftPortType=input  RightPortType=output  PseudoPeriodic=off  Frequencies=[]  VectorFormat=1-D array  Unit=kW  AffineConversion=off
  PS-Simulink Converter1 : nesl_utility/PS-Simulink Converter  PhysicalDomain=network_engine_domain  SubClassName=ps_output  LeftPortType=input  RightPortType=output  PseudoPeriodic=off  Frequencies=[]  VectorFormat=1-D array  Unit=A  AffineConversion=off
  Power Sensor : ee_lib/Sensors & Transducers/Power Sensor  measurement_type=1  averaging_period=1e-4 s
  S : PMIOPort  Side=Left
  - : PMIOPort  Port=2  Side=Left
  + : PMIOPort  Port=3  Side=Right
  tag scope: Ifc=global, Pfc=global
  wires:
  PS-Simulink Converter/1 -> [Pfc]
  PS-Simulink Converter1/1 -> [Ifc]
  connections:
  +/RConn1 -- Power Sensor/LConn2
  Power Sensor/LConn3 -- -/RConn1
  PS-Simulink Converter/LConn1 -- Power Sensor/RConn1
  PS-Simulink Converter1/LConn1 -- Current Sensor/RConn1
  Current Sensor/LConn1 -- S/RConn1
  Current Sensor/RConn2 -- Power Sensor/LConn1

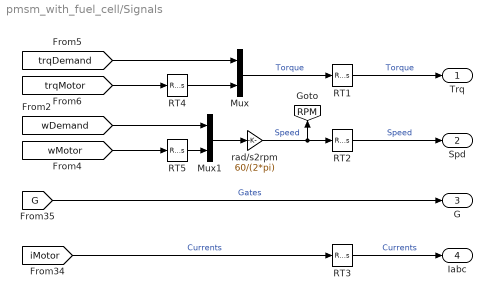
== system pmsm_with_fuel_cell/Signals  ==
  Mux : Mux  Inputs=2
  Mux1 : Mux  Inputs=2
  RT1 : RateTransition  OutPortSampleTime=Ts
  RT2 : RateTransition  OutPortSampleTime=Ts
  RT3 : RateTransition  OutPortSampleTime=Ts
  RT4 : RateTransition  OutPortSampleTime=Tsc
  RT5 : RateTransition  OutPortSampleTime=Tsc
  rad/s2rpm : Gain  Gain=60/(2*pi)
  Trq : Outport  VectorParamsAs1DForOutWhenUnconnected=off
  Spd : Outport  Port=2  VectorParamsAs1DForOutWhenUnconnected=off
  G : Outport  Port=3  VectorParamsAs1DForOutWhenUnconnected=off
  Iabc : Outport  Port=4  VectorParamsAs1DForOutWhenUnconnected=off
  tag scope: RPM=global
  wires:
  [trqDemand] -> Mux/1
  [G] -> G/1  "Gates"
  Mux1/1 -> rad/s2rpm/1
  Mux/1 -> RT1/1  "Torque"
  [iMotor] -> RT3/1  "Currents"
  [wDemand] -> Mux1/1
  rad/s2rpm/1 -> [RPM], RT2/1  "Speed"
  [trqMotor] -> RT4/1
  [wMotor] -> RT5/1
  RT1/1 -> Trq/1  "Torque"
  RT2/1 -> Spd/1  "Speed"
  RT3/1 -> Iabc/1  "Currents"
  RT4/1 -> Mux/2
  RT5/1 -> Mux1/2

== system pmsm_with_fuel_cell/Subsystem ==
  Clock : Clock
  MATLAB Function : MATLAB Function  TreatAsAtomicUnit=on
  isdone : Outport
  wires:
  [V_bus] -> MATLAB Function/1(V_bus)
  [I_fc_1] -> MATLAB Function/2(I_fc)
  [I_bat_1] -> MATLAB Function/3(I_bat)
  Clock/1 -> MATLAB Function/4(t)
  MATLAB Function/1(isdone) -> isdone/1

== system pmsm_with_fuel_cell/Subsystem2 ==
  Gain : Gain  Gain=100*(1/30)
  PS-Simulink Converter1 : nesl_utility/PS-Simulink Converter  PhysicalDomain=network_engine_domain  SubClassName=ps_output  LeftPortType=input  RightPortType=output  PseudoPeriodic=off  Frequencies=[]  VectorFormat=1-D array  Unit=A*hr  AffineConversion=off
  q : PMIOPort  Side=Left
  tag scope: Qbat=global
  wires:
  PS-Simulink Converter1/1 -> Gain/1
  Gain/1 -> [Qbat]
  connections:
  PS-Simulink Converter1/LConn1 -- q/RConn1
